simulink model "PIDtuning"  (R2026a)
settings: Solver=FixedStepAuto  StopTime=4  FixedStep=0.01
values from neighbouring files (symbols this model uses):
  Kd = 0.05    [PID_tuning.m]
  Ki = 0    [PID_tuning.m]
  Kp = 0.5    [PID_tuning.m]
libraries: arduinolib x2, simulink x1, arduinosensorlib x1, slpidlib x1
settings Model: SILPILModeSetting=veronly  ExtModeTrigDuration=2  Creator=Johannes  LastModifiedBy=Johannes
settings HardwareCC: ProdBitPerInt=16.0  ProdBitPerPointer=16.0  ProdBitPerSizeT=16.0  ProdBitPerPtrDiffT=16.0  ProdWordSize=8.0  ProdHWDeviceType=Atmel->AVR  UseEmbeddedCoderFeatures=off  UseSimulinkCoderFeatures=off
settings RTWCC: SystemTargetFile=ert.tlc  HardwareBoard=Arduino Mega 2560  TLCOptions=-aInlineSetEventsForThisBaseRateFcn=TLC_FALSE -aSuppressMultiTaskScheduler=TLC_FALSE -aRateBasedStepFcn=1  Toolchain=Arduino AVR  Description=Embedded Coder
settings CodeAppCC: MangleLength=10.0
settings ERTTargetCC: ExtModeTransport=3.0  ExtModeAutomaticAllocSize=off  ExtModeStaticAllocSize=2048.0  SupportContinuousTime=on  SupportNonInlinedSFcns=on  SupportVariableSizeSignals=on

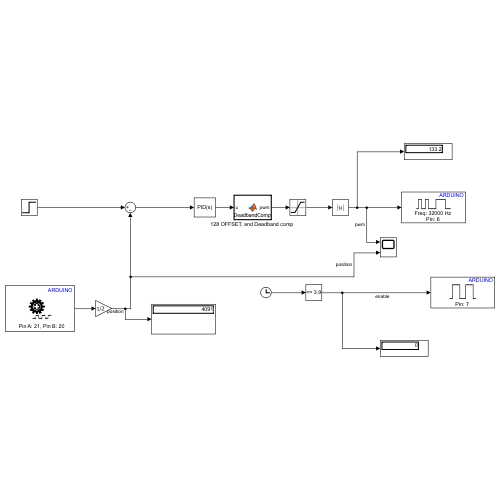
[thumbnail: Simulink's stored preview of the top-level diagram]
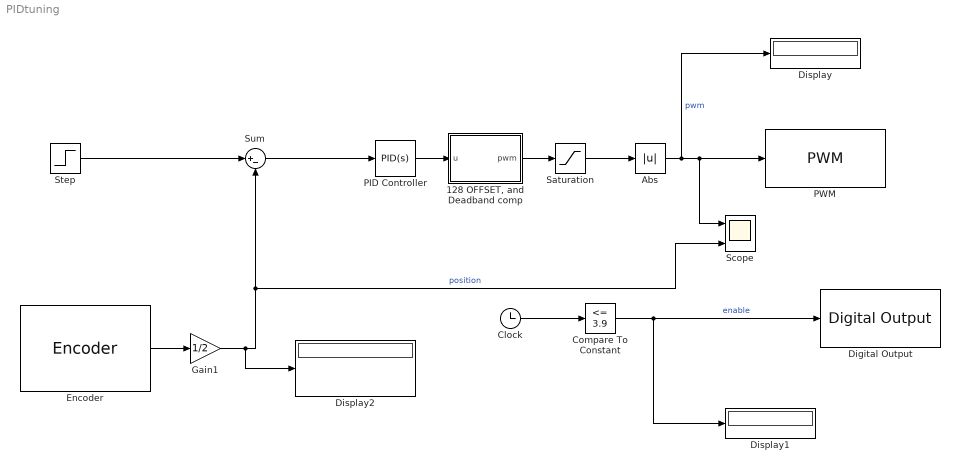
== system PIDtuning ==
  "128 OFFSET, and Deadband comp " : MATLAB Function  TreatAsAtomicUnit=on
  Abs : Abs  SaturateOnIntegerOverflow=off
  Clock : Clock
  Compare To Constant : simulink/Logic and Bit Operations/Compare To Constant  relop=<=  const=3.9  OutDataTypeStr=boolean
  Digital Output : arduinolib/Digital Output  pinNumber=7  Direction=output  blockPlatform=arduino
  Display : Display
  Display1 : Display
  Display2 : Display
  Encoder : arduinosensorlib/Encoder  InputA=21  InputB=20  Mode=No reset  SampleTime=-1
  Gain1 : Gain  Gain=1/2
  PID Controller : slpidlib/PID Controller  Controller=PID  Form=Parallel  TimeDomain=Continuous-time  UseExternalTs=off  SampleTime=-1  IntegratorMethod=Forward Euler  FilterMethod=Forward Euler  ControllerParametersSource=internal  P=Kp  I=Ki  UseKiTs=off  D=Kd  UseExternalDerivativeSource=off  N=100  UseFilter=on  TunerSelectOption=Transfer Function Based (PID Tuner App)  InitialConditionSource=internal  InitialConditionForIntegrator=0  InitialConditionForFilter=0  DifferentiatorICPrevScaledInput=0  ExternalReset=none  TrackingMode=off  Kt=1  LimitOutput=off  SatLimitsSource=internal  UpperSaturationLimit=inf  LowerSaturationLimit=-inf  LinearizeAsGain=on  AntiWindupMode=none  Kb=1  LimitIntegrator=off  UpperIntegratorSaturationLimit=inf  LowerIntegratorSaturationLimit=-inf  POutMin=[]  POutMax=[]  IOutMin=[]  IOutMax=[]  DOutMin=[]  DOutMax=[]  NOutMin=[]  NOutMax=[]  SumOutMin=[]  SumOutMax=[]  SaturationOutMin=[]  SaturationOutMax=[]  PParamMin=[]  PParamMax=[]  IParamMin=[]  IParamMax=[]  DParamMin=[]  DParamMax=[]  NParamMin=[]  NParamMax=[]  KbParamMin=[]  KbParamMax=[]  KtParamMin=[]  KtParamMax=[]  KbOutMin=[]  KbOutMax=[]  KtOutMin=[]  KtOutMax=[]  IntegratorOutMin=[]  IntegratorOutMax=[]  FilterOutMin=[]  FilterOutMax=[]  SumI1OutMin=[]  SumI1OutMax=[]  SumI2OutMin=[]  SumI2OutMax=[]  SumI3OutMin=[]  SumI3OutMax=[]  SumI4OutMin=[]  SumI4OutMax=[]  SumDOutMin=[]  SumDOutMax=[]  DifferentiatorOutMin=[]  DifferentiatorOutMax=[]  FilterDiffOutCoefMin=[]  FilterDiffOutCoefMax=[]  ReciprocalOutMin=[]  ReciprocalOutMax=[]  SumDenOutMin=[]  SumDenOutMax=[]  SumNumOutMin=[]  SumNumOutMax=[]  DivideOutMin=[]  DivideOutMax=[]  UdiffTsProdOutMin=[]  UdiffTsProdOutMax=[]  NTsProdOutMin=[]  NTsProdOutMax=[]  UintegralTsProdOutMin=[]  UintegralTsProdOutMax=[]  UngainTsProdOutMin=[]  UngainTsProdOutMax=[]  ClampingZeroOutDataTypeStr=Inherit: Inherit via back propagation  ClampingZeroOutMin=[]  ClampingZeroOutMax=[]  FilterDenConstantOutDataTypeStr=Inherit: Inherit via back propagation  FilterDenConstantOutMin=[]  FilterDenConstantOutMax=[]  PCopyOutDataTypeStr=Inherit: Inherit via back propagation  PCopyOutMin=[]  PCopyOutMax=[]  NCopyOutDataTypeStr=Inherit: Inherit via back propagation  NCopyOutMin=[]  NCopyOutMax=[]  IntegratorContinuousStateAttributes=''  IntegratorStateMustResolveToSignalObject=off  IntegratorRTWStateStorageClass=Auto  FilterContinuousStateAttributes=''  FilterStateMustResolveToSignalObject=off  FilterRTWStateStorageClass=Auto  ParallelPVariant=InternalParameters  IdealPVariant=Disabled  IVariant=InternalParameters  DVariant=InternalParameters  IntegratorVariant=Continuous  SatVariant=Disabled  AWVariant=Passthrough  PCopyVariant=Disabled  TRVariant=Disabled  FdbkBlocksVariant=Forward  IdealPFdbkVariant=Disabled  SatFdbkVariant=Disabled  DerivativeFilterVariant=ContFilter  NVariant=InternalParameters  NCopyVariant=Disabled  FilterICVariant=InternalICsFilter  IntegratorICVariant=InternalICs  ExternalResetVariant=Disabled  TRSumVariant=Passthrough  SumFdbkVariant=Disabled  SumVariant=Sum_PID  TsampFilterVariant=InternalTs  TsampNgainVariant=Passthrough  TsampIntegralVariant=Disabled_SignalSpec  ExternalSaturationOutDataTypeStr=Inherit: Same as second input  DerivativeSourceVariant=ErrorSignal  PreIntVariant=InternalPreInt
  PWM : arduinolib/PWM  pinNumber=6  frequencyType=Specify  desiredFrequency=32000  achievableFrequency=32000
  Saturation : Saturate  UpperLimit=255  LowerLimit=0
  Scope : Scope  NumInputPorts=2
      settings: ActiveDisplayYMinimum=-511.93749999999989  ActiveDisplayYMaximum=4607.4375  DataLoggingVariableName=scope
  Step : Step  Time=0  FinalValue=4096  SampleTime=0
  Sum : Sum  Inputs=|+-
  wires:
  Clock/1 -> Compare To Constant/1
  Compare To Constant/1 -> Digital Output/1, Display1/1  "enable"
  Encoder/1 -> Gain1/1
  Gain1/1 -> Scope/2, Sum/2, Display2/1  "position"
  Step/1 -> Sum/1
  PID Controller/1 -> "128 OFFSET, and Deadband comp "/1(u)
  Saturation/1 -> Abs/1
  "128 OFFSET, and Deadband comp "/1(pwm) -> Saturation/1
  Sum/1 -> PID Controller/1
  Abs/1 -> Display/1, Scope/1, PWM/1  "pwm"

== matlab function PIDtuning/128 OFFSET, and Deadband comp  ==
  data: u input; pwm output
function pwm = DeadbandComp(u)

deadbandPos = 4;
deadbandNeg = 4;

u = min(max(u, -128), 128);

if u > 0
    pwm = 128 + deadbandPos + ((127-deadbandPos)*u/256);

elseif u < 0
    pwm = 128 - deadbandNeg + (127-deadbandNeg)*u/256;

else
    pwm = 128;

end
